simulink subsystem "PieroControladoZ"  (R2022b)
settings: Solver=VariableStepAuto  StartTime=0.0  StopTime=10.0  RelTol=1e-3
settings Model: Creator=miriamfreiriasanjuan  LastModifiedBy=miriamfreiriasanjuan

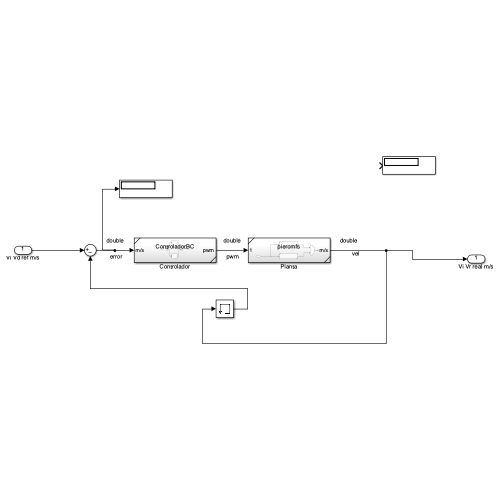
[thumbnail: Simulink's stored preview of the top-level diagram]
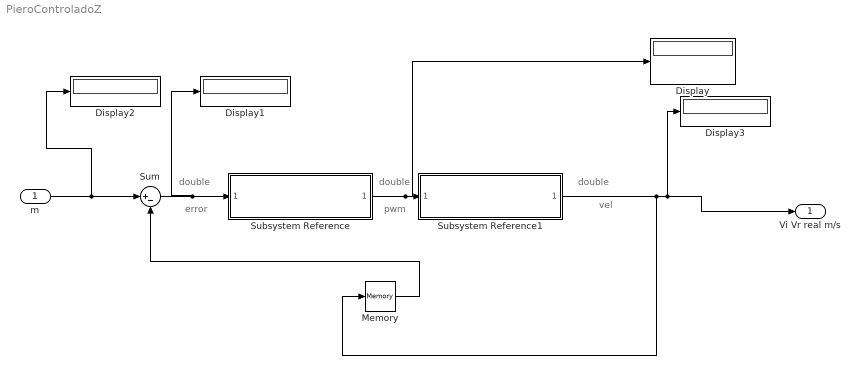
== system PieroControladoZ ==
  note: pwm
  note: double
  note: double
  note: error
  note: double
  note: vel
  m : Inport  OutDataTypeStr=double  PortDimensions=2
  Display{,1..3} (4 alike) : Display
  Memory : Memory
  Subsystem Reference : Subsystem  ReferencedSubsystem=ControladorBCz
  Subsystem Reference1 : Subsystem  ReferencedSubsystem=pieromfsZ
  Sum : Sum  Inputs=|+-
  Vi Vr real m/s : Outport
  wires:
  m/1 -> Sum/1, Display2/1
  Sum/1 -> Display1/1, Subsystem Reference/1
  Memory/1 -> Sum/2
  Subsystem Reference1/1 -> Memory/1, Vi Vr real m/s/1, Display3/1
  Subsystem Reference/1 -> Subsystem Reference1/1, Display/1
